simulink model "antenna_v5_sim"  (R2026a)
settings: Solver=FixedStepDiscrete  StopTime=48  FixedStep=1e-3
InitFcn:
  | addpath(fileparts(get_param(bdroot,'FileName')));
model workspace (MAT data in the model file):
  V5.K = [50 0.135982073305 2.1 0.0025 60 11.2 0.012 0.0001 0.002 0.05 3.8e-06 4 54.8420505496 0.0775013535651 0.00174532925199 0.00769579152915 -1.65022289217e-05 7.31427047148e-09 0.02 0.001 0.01 0.002 0.00621665704436 0.00308806936171 0.015 12 0.15 0.00349065850399 1.6 6.19120173849 0.1 200 0.496783051501]
  V5.Nr = 50
  V5.I = 1.2
  V5.ratio = 4
  V5.dout = 0.000490873852123
  V5.idle_delay = 0.3
  V5.idle_ratio = 0.5
  V5.h = 5e-05
  V5.el0 = 1.57079632679
  V5.sgn = 1
  V5.offset = 2.15373629696
  V5.a1 = 0.00872664625997
  V5.p1 = 0.523598775598
  V5.a2 = 0.00523598775598
  V5.p2 = 1.91986217719
  V5.noise = 0.000209439510239
  V5.zero = 2.15716048296
  V5.Ts = 0.00999999977648
  V5.E = 0.104719758034
  V5.V = 0.453785598278
  V5.vmax = 0.453785598278
  V5.accel = 1.04719758034
  V5.db_in = 0.000523598748259
  V5.db_out = 0.00174532923847
  V5.smooth = 13
  V5.el_init = 1.57079637051
  V5.el_min = 0.785398185253
  V5.el_max = 2.35619449615
  V5.el_rate = 0.523598790169
  V5.el_ref = 1.57079637051
  V5.us_ref = 1500
  V5.us_per_rad = 636.619750977
  V5.us_min = 1000
  V5.us_max = 2000
  az_table = [0  1.0471975512; 12  2.61799387799; 24  0.523598775598; 36  1.57079632679; 48  1.57079632679]
  el_table = [0  1.0471975512; 12  1.57079632679; 24  2.09439510239; 36  1.3962634016; 48  1.3962634016]
  fisV5 : sugfis (value not decoded)
values from neighbouring files (symbols this model uses):
  V5 = v5_simulink_params(cfg)    [v5_build_simulink.m]    (also in v5_simulink_params.m = struct(      'K', v5_plant_K(P), 'Nr', P.Nr, 'I', P.I_set, ')
libraries: fuzblock x1
settings Model: Creator=vutua  LastModifiedBy=vutua

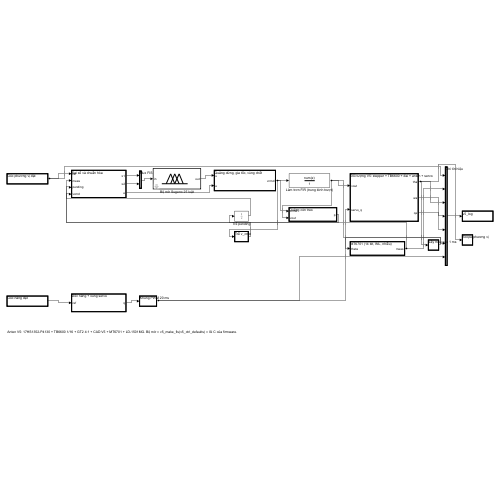
[thumbnail: Simulink's stored preview of the top-level diagram]
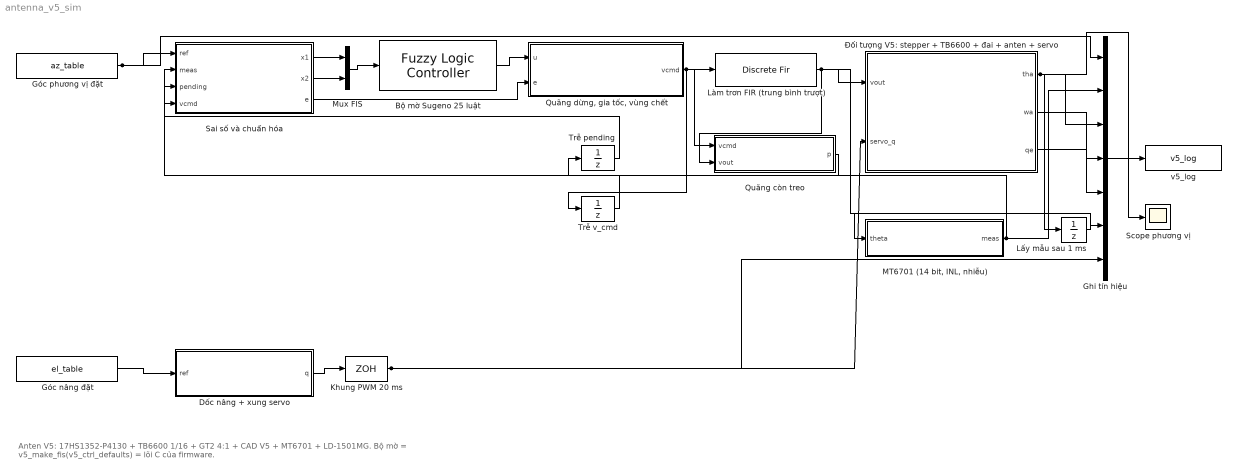
== system antenna_v5_sim ==
  note: Anten V5: 17HS1352-P4130 + TB6600 1/16 + GT2 4:1 + CAD V5 + MT6701 + LD-1501MG. Bộ mờ = v5_make_fis(v5_ctrl_defaults) = lõi C của firmware.
  Bộ mờ Sugeno 25 luật : fuzblock/Fuzzy Logic  Controller  FIS=fisV5  OutputSampleNumber=101  DataType=double  UseLookupTable=off  NumBreakpoints=10  FuzzifiedInputs=off  RuleFiringStrengths=off  RuleOutputs=off  AggregatedOutputs=off  SimulateUsing=Interpreted execution  OutOfRangeInputValueMessage=warning  NoRuleFiredMessage=warning  EmptyOutputFuzzySetMessage=warning
  Dốc nâng + xung servo : MATLAB Function  TreatAsAtomicUnit=on
  Ghi tín hiệu : Mux  Inputs=7
  Góc nâng đặt : FromWorkspace  VariableName=el_table  SampleTime=0.01  Interpolate=off  OutputAfterFinalValue=Holding final value
  Góc phương vị đặt : FromWorkspace  VariableName=az_table  SampleTime=0.01  Interpolate=off  OutputAfterFinalValue=Holding final value
  Khung PWM 20 ms : ZeroOrderHold  SampleTime=0.02
  Làm trơn FIR (trung bình trượt) : DiscreteFir  Coefficients=ones(1, V5.smooth)/V5.smooth  SampleTime=0.01
  Lấy mẫu sau 1 ms : UnitDelay  SampleTime=0.001
  "MT6701 (14 bit, INL, nhiễu)" : MATLAB Function  TreatAsAtomicUnit=on
  Mux FIS : Mux  Inputs=2
  Quãng còn treo : MATLAB Function  TreatAsAtomicUnit=on
  "Quãng dừng, gia tốc, vùng chết" : MATLAB Function  TreatAsAtomicUnit=on
  Sai số và chuẩn hóa : MATLAB Function  TreatAsAtomicUnit=on
  Scope phương vị : Scope
  Trễ pending : UnitDelay  SampleTime=0.01
  Trễ v_cmd : UnitDelay  SampleTime=0.01
  v5_log : ToWorkspace  VariableName=v5_log  SaveFormat=Structure With Time  SampleTime=-1
  Đối tượng V5: stepper + TB6600 + đai + anten + servo : MATLAB Function  TreatAsAtomicUnit=on
  wires:
  Góc phương vị đặt/1 -> Sai số và chuẩn hóa/1(ref), Ghi tín hiệu/1
  "MT6701 (14 bit, INL, nhiễu)"/1(meas) -> Sai số và chuẩn hóa/2(meas), Ghi tín hiệu/2
  Trễ pending/1 -> Sai số và chuẩn hóa/3(pending)
  Trễ v_cmd/1 -> Sai số và chuẩn hóa/4(vcmd)
  Sai số và chuẩn hóa/1(x1) -> Mux FIS/1
  Sai số và chuẩn hóa/2(x2) -> Mux FIS/2
  Mux FIS/1 -> Bộ mờ Sugeno 25 luật/1
  Bộ mờ Sugeno 25 luật/1 -> "Quãng dừng, gia tốc, vùng chết"/1(u)
  Sai số và chuẩn hóa/3(e) -> "Quãng dừng, gia tốc, vùng chết"/2(e)
  "Quãng dừng, gia tốc, vùng chết"/1(vcmd) -> Làm trơn FIR (trung bình trượt)/1, Quãng còn treo/1(vcmd), Trễ v_cmd/1
  Làm trơn FIR (trung bình trượt)/1 -> Quãng còn treo/2(vout), Đối tượng V5: stepper + TB6600 + đai + anten + servo/1(vout), Ghi tín hiệu/6
  Quãng còn treo/1(p) -> Trễ pending/1
  Góc nâng đặt/1 -> Dốc nâng + xung servo/1(ref)
  Dốc nâng + xung servo/1(q) -> Khung PWM 20 ms/1
  Khung PWM 20 ms/1 -> Đối tượng V5: stepper + TB6600 + đai + anten + servo/2(servo_q), Ghi tín hiệu/7
  Đối tượng V5: stepper + TB6600 + đai + anten + servo/1(tha) -> Lấy mẫu sau 1 ms/1, Ghi tín hiệu/3, Scope phương vị/1
  Lấy mẫu sau 1 ms/1 -> "MT6701 (14 bit, INL, nhiễu)"/1(theta)
  Đối tượng V5: stepper + TB6600 + đai + anten + servo/2(wa) -> Ghi tín hiệu/4
  Đối tượng V5: stepper + TB6600 + đai + anten + servo/3(qe) -> Ghi tín hiệu/5
  Ghi tín hiệu/1 -> v5_log/1

== matlab function antenna_v5_sim/Sai số và chuẩn hóa ==
  settings: updateMethod=DISCRETE  sampleTime=0.01
  data: ref input; x1 output; meas input; pending input; vcmd input; x2 output; e output; V5 parameter
function [x1, x2, e] = norm_in(ref, meas, pending, vcmd, V5)
e = ref - (meas + pending);
x1 = min(1, max(-1, e/V5.E));
x2 = min(1, max(-1, -vcmd/V5.V));

== matlab function antenna_v5_sim/MT6701 (14 bit, INL, nhiễu) ==
  settings: updateMethod=DISCRETE  sampleTime=0.01
  data: theta input; meas output; V5 parameter
function meas = mt6701(theta, V5)
phi = V5.sgn*theta + V5.offset;
e = V5.a1*sin(phi + V5.p1) + V5.a2*sin(2*phi + V5.p2);
raw = mod(round((phi + e + V5.noise*randn)*16384/(2*pi)), 16384);
d = mod(raw*2*pi/16384 - V5.zero + pi, 2*pi) - pi;
meas = V5.sgn*d;

== matlab function antenna_v5_sim/Quãng dừng, gia tốc, vùng chết ==
  settings: updateMethod=DISCRETE  sampleTime=0.01
  data: u input; vcmd output; e input; V5 parameter
function vcmd = governor(u, e, V5)
persistent v settled
if isempty(v), v = 0; settled = true; end
ae = abs(e);
if settled
  if ae > V5.db_out, settled = false; end
elseif ae < V5.db_in
  settled = true;
end
if settled
  vd = 0;
else
  vd = V5.vmax*u;
  h = 0.5*V5.accel*V5.Ts; vb = sqrt(h*h + 2*V5.accel*ae) - h;
  vd = min(vb, max(-vb, vd));
end
v = v + min(V5.accel*V5.Ts, max(-V5.accel*V5.Ts, vd - v));
vcmd = v;

== matlab function antenna_v5_sim/Quãng còn treo ==
  settings: updateMethod=DISCRETE  sampleTime=0.01
  data: vcmd input; p output; vout input; V5 parameter
function p = pending(vcmd, vout, V5)
persistent acc
if isempty(acc), acc = 0; end
acc = acc + (vcmd - vout)*V5.Ts;
p = acc;

== matlab function antenna_v5_sim/Dốc nâng + xung servo ==
  settings: updateMethod=DISCRETE  sampleTime=0.01
  data: ref input; q output; V5 parameter
function q = elevation(ref, V5)
persistent c
if isempty(c), c = V5.el_init; end
r = min(V5.el_max, max(V5.el_min, ref));
c = c + min(V5.el_rate*V5.Ts, max(-V5.el_rate*V5.Ts, r - c));
us = round(min(V5.us_max, max(V5.us_min, V5.us_ref + (c - V5.el_ref)*V5.us_per_rad)));
q = (us - 500)/2000*pi;

== matlab function antenna_v5_sim/Đối tượng V5: stepper + TB6600 + đai + anten + servo ==
  settings: updateMethod=DISCRETE  sampleTime=0.001
  data: vout input; tha output; servo_q input; wa output; qe output; V5 parameter
function [tha, wa, qe] = plant(vout, servo_q, V5)
persistent x acc cnt tlast t
if isempty(x)
  x = zeros(9,1); x(3) = V5.I; x(7) = V5.el0;
  acc = 0; cnt = 0; t = 0; tlast = 0;
end
h = V5.h; n = round(0.001/h);
for s = 1:n
  acc = acc + vout*h;
  c2 = round(acc/V5.dout);
  if c2 ~= cnt, cnt = c2; tlast = t; end
  thc = cnt*V5.dout*V5.ratio;
  I = V5.I; if t - tlast > V5.idle_delay, I = I*V5.idle_ratio; end
  U = [I*cos(V5.Nr*thc), I*sin(V5.Nr*thc), servo_q, 0, 0, 0];
  k1 = v5_plant_rhs(x, V5.K, U);
  k2 = v5_plant_rhs(x + 0.5*h*k1, V5.K, U);
  k3 = v5_plant_rhs(x + 0.5*h*k2, V5.K, U);
  k4 = v5_plant_rhs(x + h*k3, V5.K, U);
  x = x + h/6*(k1 + 2*k2 + 2*k3 + k4);
  t = t + h;
end
tha = x(5); wa = x(6); qe = x(7);
